simulink model "TFeteBusSrvo"  (R2025a)
settings: Solver=ode4  StartTime=0.0  StopTime=10.0  FixedStep=0.01  RelTol=1e-3
undefined symbols (not defined in the file or in its folder): RS422, TTL, UART4, UART5
libraries: AFCToolbox x5, simulink x5, etargetslib x5
settings Model: Creator=zqinghua  LastModifiedBy=zqhkd
settings OptimizationCC: DefaultParameterBehavior=Inlined  EnhancedBackFolding=on  PassReuseOutputArgsAs=Individual arguments  ZeroExternalMemoryAtStartup=off  ZeroInternalMemoryAtStartup=off  OptimizeBlockOrder=speed  DifferentSizesBufferReuse=on  OptimizationCustomize=off  EfficientTunableParamExpr=on
settings DebuggingCC: ParameterTunabilityLossMsg=error
settings HardwareCC: ProdBitPerInt=16.0  ProdBitPerPointer=16.0  ProdBitPerSizeT=16.0  ProdBitPerPtrDiffT=16.0  ProdLargestAtomicFloat=None  ProdWordSize=16.0  ProdHWDeviceType=STMicroelectronics->ST10/Super10
settings SFSimCC: MATLABDynamicMemAlloc=off
settings RTWCC: SystemTargetFile=AFCHawk.tlc  GenCodeOnly=on  TemplateMakefile=ert_default_tmf  GPUComputeCapability=3.5  Description=Embedded Coder
settings CodeAppCC: ForceParamTrailComments=on  IgnoreCustomStorageClasses=off  OperatorAnnotations=on  SimulinkDataObjDesc=on  SFDataObjDesc=on  InsertBlockDesc=on
settings STFCustomTargetCC: SystemTargetFile=AFCHawk.tlc  TargetLangStandard=C99 (ISO)  MultiwordLength=256.0  DynamicStringBufferSize=256.0  ModelReferenceCompliant=off  CombineOutputUpdateFcns=on  ERTCustomFileBanners=on  SupportContinuousTime=off  SupportNonInlinedSFcns=off  RemoveResetFunc=on  MATLABClassNameForMDSCustomization=Simulink.SoftwareTarget.ERTCustomization  GRTInterface=off  t_BuildCPrj2Hex=on  t_comBaud=460800.0  t_productKey=45638.0  t_productId=1.0  t_DownLoad2Target=on  t_comPort=2.0  t_userCode=11120.0
settings ERTTargetCC: ExtModeTransport=0.0  ExtModeStaticAlloc=off  ExtModeMexFile=ext_comm  ExtModeIntrfLevel=Level1  ERTCustomFileTemplate=example_file_process.tlc  DynamicArrayContainerType=coder::array  TargetLangStandard=C99 (ISO)  ModelReferenceCompliant=off  ParMdlRefBuildCompliant=off  CompOptLevelCompliant=off  ConcurrentExecutionCompliant=off  ModelStepFunctionPrototypeControlCompliant=off  CPPClassGenCompliant=off  UseToolchainInfoCompliant=off

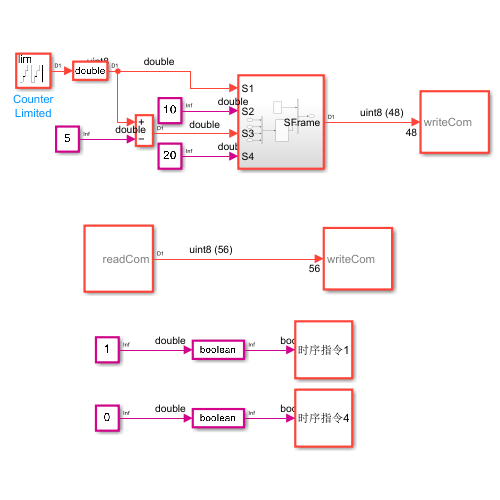
[thumbnail: Simulink's stored preview of the top-level diagram]
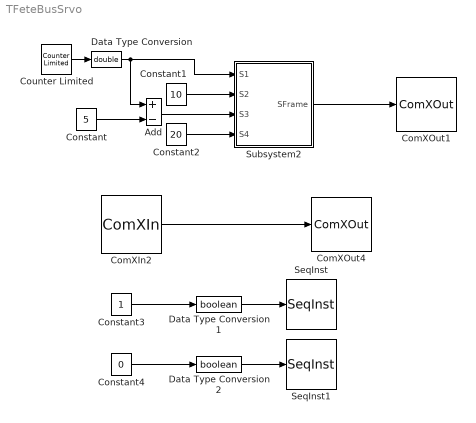
== system TFeteBusSrvo ==
  Add : Sum  Inputs=+-
  ComXIn2 : AFCToolbox/DeviceModule/ComXIn  Priority=2  g_sampleTime=0.01  g_comPort=UART4(TTL)  g_baudRate=1000000  g_dataSize=56  g_parity=0  g_stopBits=1
      settings: SourceProductName=AFCToolbox
  ComXOut1 : AFCToolbox/DeviceModule/ComXOut  Priority=8  g_comPort=UART4(TTL)  g_baudRate=1000000  g_outFreq=100
      settings: SourceProductName=AFCToolbox
  ComXOut4 : AFCToolbox/DeviceModule/ComXOut  Priority=8  g_comPort=UART5(RS422)  g_baudRate=460800  g_outFreq=1
      settings: SourceProductName=AFCToolbox
  Constant : Constant  Value=5
  Constant1 : Constant  Value=10
  Constant2 : Constant  Value=20
  Constant3 : Constant
  Constant4 : Constant  Value=0
  Counter Limited : simulink/Sources/Counter Limited  uplimit=30  tsamp=-1
  Data Type Conversion : DataTypeConversion  OutDataTypeStr=double  SaturateOnIntegerOverflow=off  RndMeth=Floor
  Data Type Conversion1 : DataTypeConversion  OutDataTypeStr=boolean  SaturateOnIntegerOverflow=off  RndMeth=Floor
  Data Type Conversion2 : DataTypeConversion  OutDataTypeStr=boolean  SaturateOnIntegerOverflow=off  RndMeth=Floor
  SeqInst : AFCToolbox/DeviceModule/SeqInst  Priority=6  g_chanelNo=时序指令1  g_comPort=0  g_instName=0  g_id=0
      settings: SourceProductName=AFCToolbox
  SeqInst1 : AFCToolbox/DeviceModule/SeqInst  Priority=6  g_chanelNo=时序指令4  g_comPort=0  g_instName=0  g_id=0
      settings: SourceProductName=AFCToolbox
  Subsystem2 : Subsystem
  wires:
  ComXIn2/1 -> ComXOut4/1
  Subsystem2/1(SFrame) -> ComXOut1/1
  Counter Limited/1 -> Data Type Conversion/1
  Constant/1 -> Add/2
  Add/1 -> Subsystem2/3(S3)
  Constant1/1 -> Subsystem2/2(S2)
  Constant2/1 -> Subsystem2/4(S4)
  Data Type Conversion/1 -> Add/1, Subsystem2/1(S1)
  Constant3/1 -> Data Type Conversion1/1
  Constant4/1 -> Data Type Conversion2/1
  Data Type Conversion1/1 -> SeqInst/1
  Data Type Conversion2/1 -> SeqInst1/1

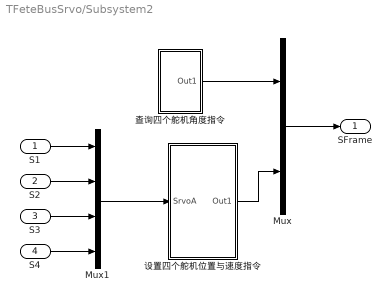
== system TFeteBusSrvo/Subsystem2 ==
  S1 : Inport
  S2 : Inport  Port=2
  S3 : Inport  Port=3
  S4 : Inport  Port=4
  Mux : Mux  Inputs=2
  Mux1 : Mux
  查询四个舵机角度指令 : Subsystem
  设置四个舵机位置与速度指令 : Subsystem
  SFrame : Outport
  wires:
  设置四个舵机位置与速度指令/1(Out1) -> Mux/2
  查询四个舵机角度指令/1(Out1) -> Mux/1
  Mux/1 -> SFrame/1
  S1/1 -> Mux1/1
  S2/1 -> Mux1/2
  S3/1 -> Mux1/3
  S4/1 -> Mux1/4
  Mux1/1 -> 设置四个舵机位置与速度指令/1(SrvoA)

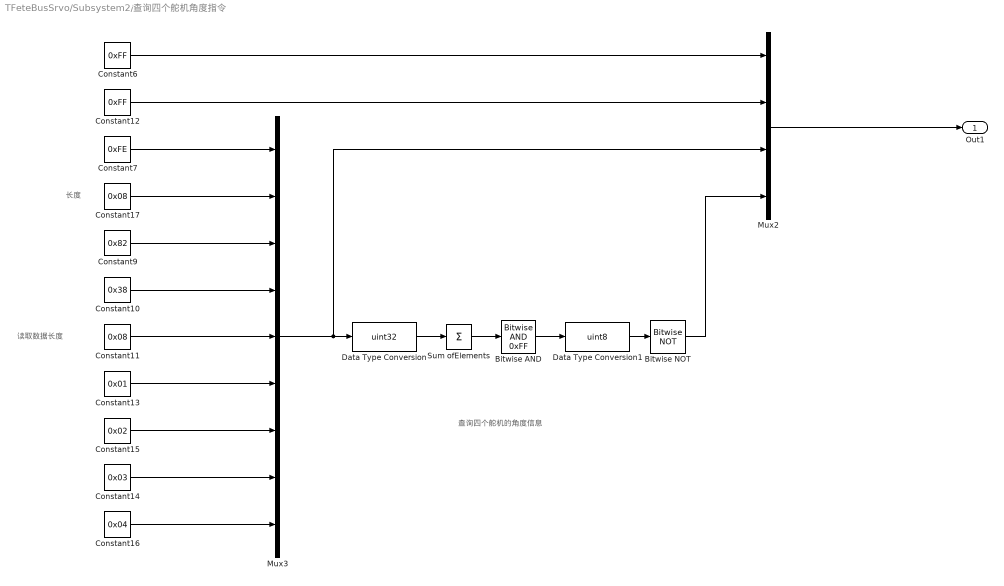
== system TFeteBusSrvo/Subsystem2/查询四个舵机角度指令 ==
  note: 查询四个舵机的角度信息
  note: 长度
  note: 读取数据长度
  Bitwise AND : simulink/Logic and Bit Operations/Bitwise Operator  logicop=AND  UseBitMask=on  BitMask=0xFF  BitMaskRealWorld=Stored Integer
      settings: LibrarySourceBlock=|
      | simulink/Quick Insert/Logic and Bit
      | Operations/Bitwise AND
  Bitwise NOT : simulink/Logic and Bit Operations/Bitwise Operator  logicop=NOT  UseBitMask=off  BitMask=bin2dec('11011001')  BitMaskRealWorld=Stored Integer
      settings: LibrarySourceBlock=|
      | simulink/Quick Insert/Logic and Bit
      | Operations/Bitwise NOT
  Constant10 : Constant  Value=0x38  OutDataTypeStr=uint8
  Constant11 : Constant  Value=0x08  OutDataTypeStr=uint8
  Constant12 : Constant  Value=0xFF  OutDataTypeStr=uint8
  Constant13 : Constant  Value=0x01
  Constant14 : Constant  Value=0x03
  Constant15 : Constant  Value=0x02
  Constant16 : Constant  Value=0x04
  Constant17 : Constant  Value=0x08  OutDataTypeStr=uint8
  Constant6 : Constant  Value=0xFF  OutDataTypeStr=uint8
  Constant7 : Constant  Value=0xFE  OutDataTypeStr=uint8
  Constant9 : Constant  Value=0x82  OutDataTypeStr=uint8
  Data Type Conversion : DataTypeConversion  OutDataTypeStr=uint32  SaturateOnIntegerOverflow=off  RndMeth=Floor
  Data Type Conversion1 : DataTypeConversion  OutDataTypeStr=uint8  SaturateOnIntegerOverflow=off  RndMeth=Floor
  Mux2 : Mux
  Mux3 : Mux  Inputs=9
  Sum ofElements : Sum  Inputs=+
  Out1 : Outport
  wires:
  Constant16/1 -> Mux3/9
  Mux3/1 -> Data Type Conversion/1, Mux2/3
  Bitwise AND/1 -> Data Type Conversion1/1
  Data Type Conversion1/1 -> Bitwise NOT/1
  Constant17/1 -> Mux3/2
  Mux2/1 -> Out1/1
  Constant12/1 -> Mux2/2
  Data Type Conversion/1 -> Sum ofElements/1
  Sum ofElements/1 -> Bitwise AND/1
  Constant14/1 -> Mux3/8
  Constant6/1 -> Mux2/1
  Constant13/1 -> Mux3/6
  Constant15/1 -> Mux3/7
  Constant10/1 -> Mux3/4
  Constant11/1 -> Mux3/5
  Bitwise NOT/1 -> Mux2/4
  Constant7/1 -> Mux3/1
  Constant9/1 -> Mux3/3

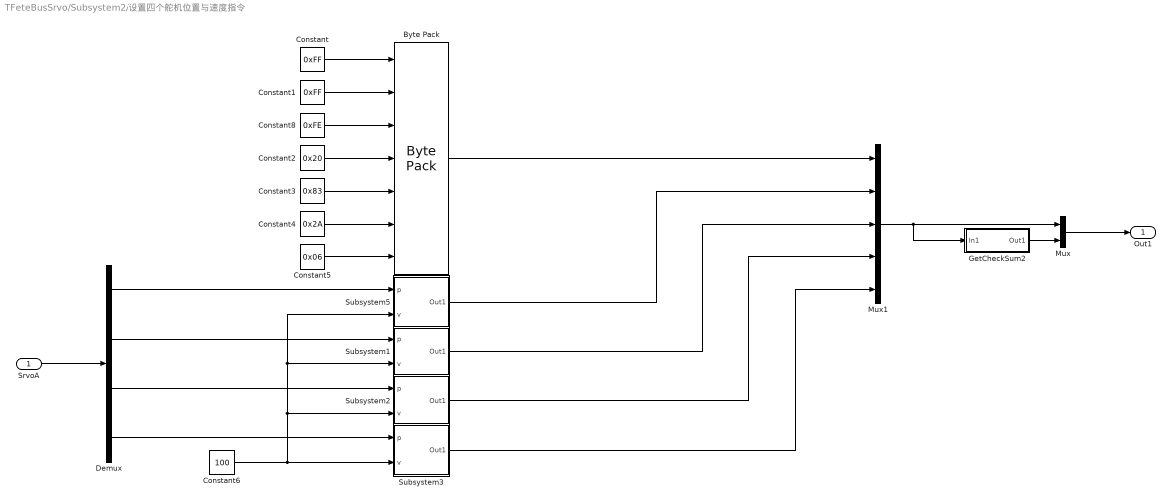
== system TFeteBusSrvo/Subsystem2/设置四个舵机位置与速度指令 ==
  SrvoA : Inport
  Byte Pack : etargetslib/Byte Pack  datatypes={'uint8','uint8','uint8','uint8','uint8','uint8','uint8'}  byteAlign=1
  Constant : Constant  Value=0xFF  OutDataTypeStr=uint8
  Constant1 : Constant  Value=0xFF  OutDataTypeStr=uint8
  Constant2 : Constant  Value=0x20  OutDataTypeStr=uint8
  Constant3 : Constant  Value=0x83  OutDataTypeStr=uint8
  Constant4 : Constant  Value=0x2A  OutDataTypeStr=uint8
  Constant5 : Constant  Value=0x06  OutDataTypeStr=uint8
  Constant6 : Constant  Value=100  OutDataTypeStr=uint8
  Constant8 : Constant  Value=0xFE  OutDataTypeStr=uint8
  Demux : Demux
  GetCheckSum2 : Subsystem
  Mux : Mux  Inputs=2
  Mux1 : Mux  Inputs=5
  Subsystem1 : Subsystem  mask{id=2}
      mask DialogControl ParameterGroupVar Prompt: id
  Subsystem2 : Subsystem  mask{id=3}
      mask DialogControl ParameterGroupVar Prompt: id
  Subsystem3 : Subsystem  mask{id=4}
      mask DialogControl ParameterGroupVar Prompt: id
  Subsystem5 : Subsystem  mask{id=1}
      mask DialogControl ParameterGroupVar Prompt: id
  Out1 : Outport
  wires:
  Mux/1 -> Out1/1
  Constant4/1 -> Byte Pack/6
  Subsystem5/1(Out1) -> Mux1/2
  Mux1/1 -> Mux/1, GetCheckSum2/1(In1)
  GetCheckSum2/1(Out1) -> Mux/2
  Constant5/1 -> Byte Pack/7
  Constant2/1 -> Byte Pack/4
  Constant1/1 -> Byte Pack/2
  Constant/1 -> Byte Pack/1
  Constant3/1 -> Byte Pack/5
  Constant8/1 -> Byte Pack/3
  Constant6/1 -> Subsystem5/2(v), Subsystem1/2(v), Subsystem2/2(v), Subsystem3/2(v)
  Byte Pack/1 -> Mux1/1
  Subsystem3/1(Out1) -> Mux1/5
  Subsystem2/1(Out1) -> Mux1/4
  Subsystem1/1(Out1) -> Mux1/3
  SrvoA/1 -> Demux/1
  Demux/1 -> Subsystem5/1(p)
  Demux/2 -> Subsystem1/1(p)
  Demux/3 -> Subsystem2/1(p)
  Demux/4 -> Subsystem3/1(p)

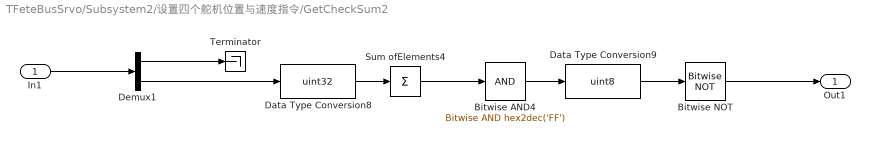
== system TFeteBusSrvo/Subsystem2/设置四个舵机位置与速度指令/GetCheckSum2 ==
  In1 : Inport
  Bitwise AND4 : simulink/Logic and Bit Operations/Bitwise Operator  logicop=AND  UseBitMask=on  BitMask=hex2dec('FF')  BitMaskRealWorld=Stored Integer
      settings: LibrarySourceBlock=|
      | simulink/Quick Insert/Logic and Bit
      | Operations/Bitwise AND
  Bitwise NOT : simulink/Logic and Bit Operations/Bitwise Operator  logicop=NOT  UseBitMask=off  BitMask=bin2dec('11011001')  BitMaskRealWorld=Stored Integer
      settings: LibrarySourceBlock=|
      | simulink/Quick Insert/Logic and Bit
      | Operations/Bitwise NOT
  Data Type Conversion8 : DataTypeConversion  OutDataTypeStr=uint32  SaturateOnIntegerOverflow=off  RndMeth=Floor
  Data Type Conversion9 : DataTypeConversion  OutDataTypeStr=uint8  SaturateOnIntegerOverflow=off  RndMeth=Floor
  Demux1 : Demux  Outputs=[2,-1]
  Sum ofElements4 : Sum  Inputs=+
  Terminator : Terminator
  Out1 : Outport
  wires:
  Data Type Conversion9/1 -> Bitwise NOT/1
  Data Type Conversion8/1 -> Sum ofElements4/1
  Sum ofElements4/1 -> Bitwise AND4/1
  Bitwise AND4/1 -> Data Type Conversion9/1
  Demux1/2 -> Data Type Conversion8/1
  Demux1/1 -> Terminator/1
  In1/1 -> Demux1/1
  Bitwise NOT/1 -> Out1/1

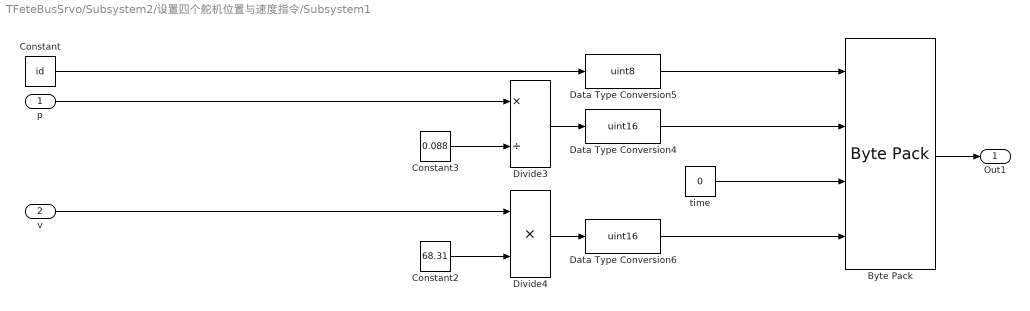
== system TFeteBusSrvo/Subsystem2/设置四个舵机位置与速度指令/Subsystem1 ==
  p : Inport
  v : Inport  Port=2
  Byte Pack : etargetslib/Byte Pack  datatypes={'uint8','uint16','uint16','uint16'}  byteAlign=1
  Constant : Constant  Value=id
  Constant2 : Constant  Value=68.31  OutDataTypeStr=double
  Constant3 : Constant  Value=0.088  OutDataTypeStr=double
  Data Type Conversion4 : DataTypeConversion  OutDataTypeStr=uint16  SaturateOnIntegerOverflow=off  RndMeth=Floor
  Data Type Conversion5 : DataTypeConversion  OutDataTypeStr=uint8  SaturateOnIntegerOverflow=off  RndMeth=Floor
  Data Type Conversion6 : DataTypeConversion  OutDataTypeStr=uint16  SaturateOnIntegerOverflow=off  RndMeth=Floor
  Divide3 : Product  Inputs=*/
  Divide4 : Product  Inputs=**
  time : Constant  Value=0  OutDataTypeStr=uint16
  Out1 : Outport
  wires:
  Byte Pack/1 -> Out1/1
  Constant/1 -> Data Type Conversion5/1
  p/1 -> Divide3/1
  Data Type Conversion5/1 -> Byte Pack/1
  v/1 -> Divide4/1
  time/1 -> Byte Pack/3
  Divide4/1 -> Data Type Conversion6/1
  Data Type Conversion4/1 -> Byte Pack/2
  Constant3/1 -> Divide3/2
  Constant2/1 -> Divide4/2
  Data Type Conversion6/1 -> Byte Pack/4
  Divide3/1 -> Data Type Conversion4/1

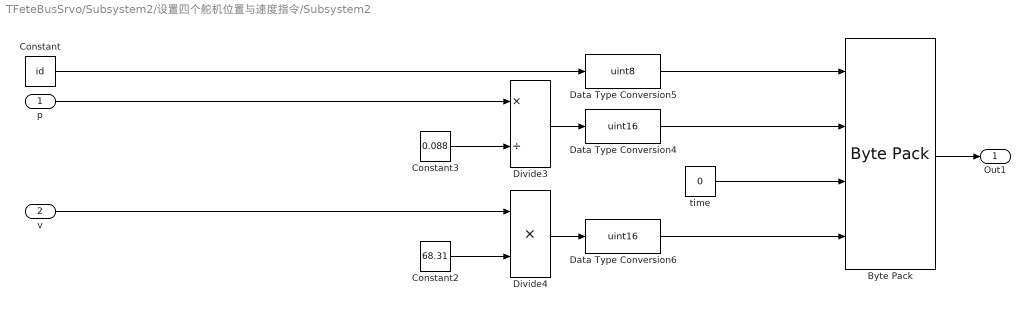
== system TFeteBusSrvo/Subsystem2/设置四个舵机位置与速度指令/Subsystem2 ==
  p : Inport
  v : Inport  Port=2
  Byte Pack : etargetslib/Byte Pack  datatypes={'uint8','uint16','uint16','uint16'}  byteAlign=1
  Constant : Constant  Value=id
  Constant2 : Constant  Value=68.31  OutDataTypeStr=double
  Constant3 : Constant  Value=0.088  OutDataTypeStr=double
  Data Type Conversion4 : DataTypeConversion  OutDataTypeStr=uint16  SaturateOnIntegerOverflow=off  RndMeth=Floor
  Data Type Conversion5 : DataTypeConversion  OutDataTypeStr=uint8  SaturateOnIntegerOverflow=off  RndMeth=Floor
  Data Type Conversion6 : DataTypeConversion  OutDataTypeStr=uint16  SaturateOnIntegerOverflow=off  RndMeth=Floor
  Divide3 : Product  Inputs=*/
  Divide4 : Product  Inputs=**
  time : Constant  Value=0  OutDataTypeStr=uint16
  Out1 : Outport
  wires:
  Divide3/1 -> Data Type Conversion4/1
  Data Type Conversion6/1 -> Byte Pack/4
  Constant2/1 -> Divide4/2
  Constant3/1 -> Divide3/2
  Data Type Conversion4/1 -> Byte Pack/2
  Divide4/1 -> Data Type Conversion6/1
  time/1 -> Byte Pack/3
  v/1 -> Divide4/1
  Data Type Conversion5/1 -> Byte Pack/1
  p/1 -> Divide3/1
  Constant/1 -> Data Type Conversion5/1
  Byte Pack/1 -> Out1/1

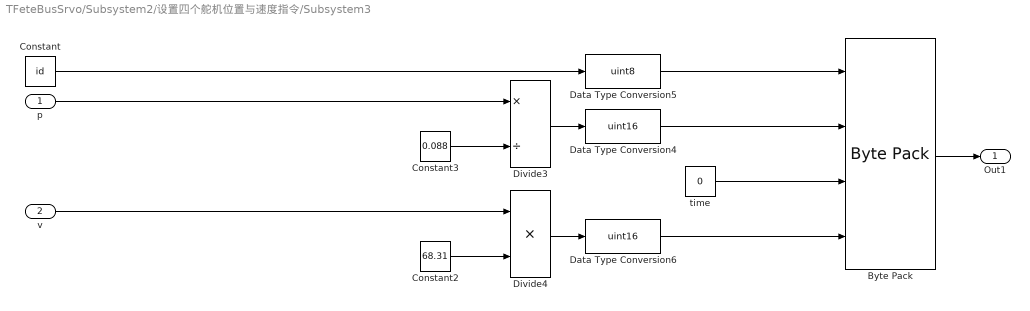
== system TFeteBusSrvo/Subsystem2/设置四个舵机位置与速度指令/Subsystem3 ==
  p : Inport
  v : Inport  Port=2
  Byte Pack : etargetslib/Byte Pack  datatypes={'uint8','uint16','uint16','uint16'}  byteAlign=1
  Constant : Constant  Value=id
  Constant2 : Constant  Value=68.31  OutDataTypeStr=double
  Constant3 : Constant  Value=0.088  OutDataTypeStr=double
  Data Type Conversion4 : DataTypeConversion  OutDataTypeStr=uint16  SaturateOnIntegerOverflow=off  RndMeth=Floor
  Data Type Conversion5 : DataTypeConversion  OutDataTypeStr=uint8  SaturateOnIntegerOverflow=off  RndMeth=Floor
  Data Type Conversion6 : DataTypeConversion  OutDataTypeStr=uint16  SaturateOnIntegerOverflow=off  RndMeth=Floor
  Divide3 : Product  Inputs=*/
  Divide4 : Product  Inputs=**
  time : Constant  Value=0  OutDataTypeStr=uint16
  Out1 : Outport
  wires:
  Byte Pack/1 -> Out1/1
  Constant/1 -> Data Type Conversion5/1
  p/1 -> Divide3/1
  Data Type Conversion5/1 -> Byte Pack/1
  v/1 -> Divide4/1
  time/1 -> Byte Pack/3
  Divide4/1 -> Data Type Conversion6/1
  Data Type Conversion4/1 -> Byte Pack/2
  Constant3/1 -> Divide3/2
  Constant2/1 -> Divide4/2
  Data Type Conversion6/1 -> Byte Pack/4
  Divide3/1 -> Data Type Conversion4/1

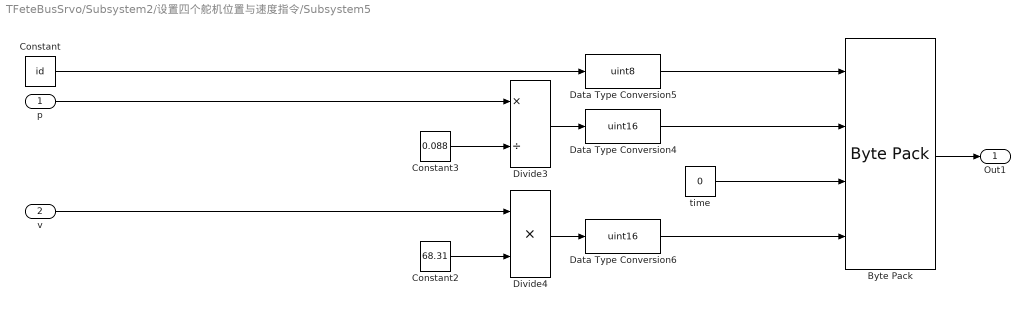
== system TFeteBusSrvo/Subsystem2/设置四个舵机位置与速度指令/Subsystem5 ==
  p : Inport
  v : Inport  Port=2
  Byte Pack : etargetslib/Byte Pack  datatypes={'uint8','uint16','uint16','uint16'}  byteAlign=1
  Constant : Constant  Value=id
  Constant2 : Constant  Value=68.31  OutDataTypeStr=double
  Constant3 : Constant  Value=0.088  OutDataTypeStr=double
  Data Type Conversion4 : DataTypeConversion  OutDataTypeStr=uint16  SaturateOnIntegerOverflow=off  RndMeth=Floor
  Data Type Conversion5 : DataTypeConversion  OutDataTypeStr=uint8  SaturateOnIntegerOverflow=off  RndMeth=Floor
  Data Type Conversion6 : DataTypeConversion  OutDataTypeStr=uint16  SaturateOnIntegerOverflow=off  RndMeth=Floor
  Divide3 : Product  Inputs=*/
  Divide4 : Product  Inputs=**
  time : Constant  Value=0  OutDataTypeStr=uint16
  Out1 : Outport
  wires:
  Divide3/1 -> Data Type Conversion4/1
  Data Type Conversion6/1 -> Byte Pack/4
  Constant2/1 -> Divide4/2
  Constant3/1 -> Divide3/2
  Data Type Conversion4/1 -> Byte Pack/2
  Divide4/1 -> Data Type Conversion6/1
  time/1 -> Byte Pack/3
  v/1 -> Divide4/1
  Data Type Conversion5/1 -> Byte Pack/1
  p/1 -> Divide3/1
  Constant/1 -> Data Type Conversion5/1
  Byte Pack/1 -> Out1/1
